simulink library "lib_AC_DFIG"  (R2026a)
settings: Solver=VariableStepAuto
undefined symbols (not defined in the file): block_buses, block_idx, buses_lf, fref, Lbiginv, Lrr_pu, Lss_pu, Nbuses, op_DFIG, Ps_lf, sigma
settings Model: Creator=atomas  LastModifiedBy=atomas

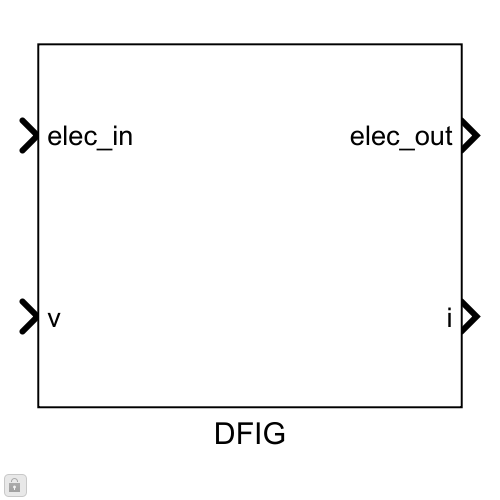
[thumbnail: Simulink's stored preview of the top-level diagram]
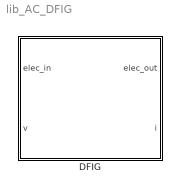
== system lib_AC_DFIG ==
  DFIG : Subsystem  mask(Doubly Fed Induction Generator){DFIGs_nodes=1, FBASE=50, D=0, H=3.3, Ls_pu=0.1178, Rs_pu=0.00734, Lm_pu=4.709, Rr_pu=0.01225, Lr_pu=0.15349, Ra_pu=0.1, La_pu=1, Cf_pu=0.0555, Ki_ia=7162, Kp_ia=6.5, Ki_ir=2117, Kp_ir=1.96, Ki_vc2=-562.5, Kp_vc2=-5.25, Ki_s=12000, Kp_s=1200, Kp_pll=2.33, Ki_pll=877}
      mask prompts: FBASE "Base frequency (Hz)"; D "Damping (pu)"; H "Inertia (s)"; Ls_pu "Stator inductances (pu)"; Rs_pu "Stator resistances (pu)"; Lm_pu "Mutual inductance (pu)"; Rr_pu "Rotor Resistance (pu)"; Lr_pu "Rotor Inductance"; Ra_pu "Filter Resistance (pu)"; La_pu "Filter Inductance (pu)"; Cf_pu "DC-Link Capacitance"; Ki_ia "GSC Ki"; Kp_ia "GSC Kp"; Ki_ir "RSC Ki"; Kp_ir "RSC Kp"; Ki_vc2 "DC Link Voltage Control Ki"; Kp_vc2 "DC Link Voltage Control Kp"; Ki_s "Slip Control Ki"; Kp_s "Slip Control Kp"; Kp_pll "PLL Kp"; Ki_pll "PLL Ki"
      mask help: Doubly Fed Induction Generator modelled in d-q reference frame.
      mask init:
      | [block_buses, block_idx, block_toM, block_fref, Lbiginv, Ls_pu, Lr_pu, Lm_pu, La_pu, Lss_pu, Lrr_pu, sigma, omega_base] = mask_init_DFIG(gcb, FBASE, Ls_pu, Lr_pu, Lm_pu, La_pu);
      mask Help: web([extractBefore(get_param(bdroot, 'filename'),gcs) 'Documentation/SM.html'])
      mask DialogControl Params Prompt: Parameters
      mask DialogControl Container10 Prompt: PI Parameters
      mask DialogControl Params_copy Prompt: Parameters

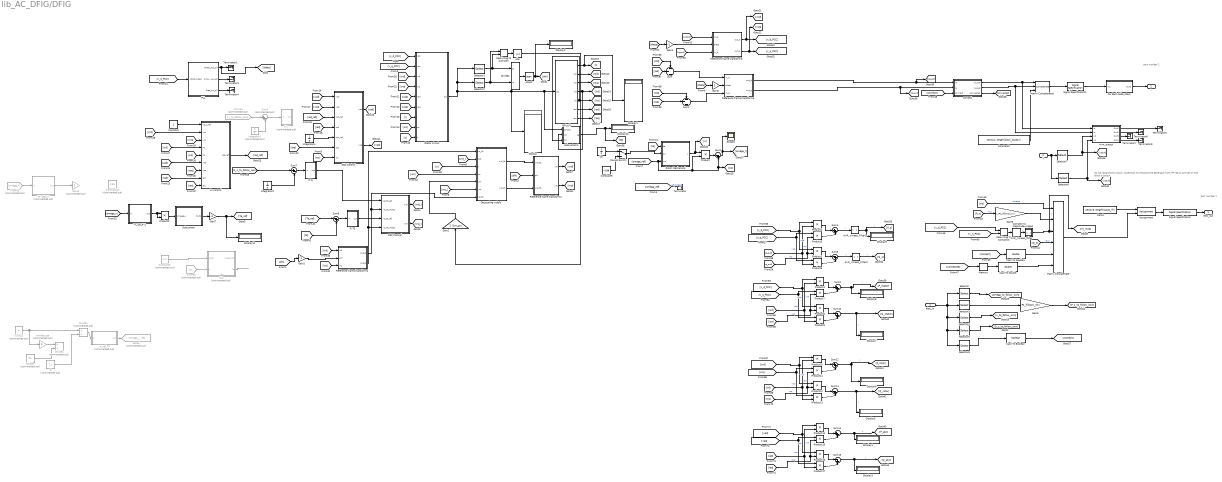
== system lib_AC_DFIG/DFIG ==
  note: do not rename this block, conditions to initialise the generator from PF result are set on this block's output
  note: port number 1
  note: port number 2
  elec_in : Inport
  v : Inport  Port=2
  AVR_Vmeas_Filter : Subsystem  mask{T_r=1e-6}
      mask prompts: T_r "Filter time constant"
      mask Display:
      | try
      |     dpoly(1, [T_r, 1])
      | catch
      | end
  AVR_Vmeas_Filter1 : Subsystem  mask{T_r=1e-6}
      mask prompts: T_r "Filter time constant"
      mask Display:
      | try
      |     dpoly(1, [T_r, 1])
      | catch
      | end
  AVR_Vmeas_Filter2 : Subsystem  mask{T_r=1e-6}
      mask prompts: T_r "Filter time constant"
      mask Display:
      | try
      |     dpoly(1, [T_r, 1])
      | catch
      | end
  Abs : Abs  SaturateOnIntegerOverflow=off
  Assignment : Assignment  NumberOfDimensions=2  DiagnosticForDimensions=Warning  IndexOptions=Assign all,Index vector (dialog)  Indices=1,block_idx  OutputSizes=1,1
  Atan2 : Trigonometry  SCDEnableBlockLinearizationSpecification=on  Operator=atan
  Cast To Boolean : DataTypeConversion  OutDataTypeStr=boolean  SaturateOnIntegerOverflow=off  RndMeth=Floor
  Cast To Double : DataTypeConversion  OutDataTypeStr=double  SaturateOnIntegerOverflow=off  RndMeth=Floor
  Cast To Double1 : DataTypeConversion  OutDataTypeStr=double  SaturateOnIntegerOverflow=off  RndMeth=Floor
  Complex to Magnitude-Angle1 : ComplexToMagnitudeAngle  Output=Magnitude
  Constant : Constant
  Constant10 : Constant  Commented=on  Value=1.83
  Constant2 : Constant  Value=zeros(1, length(block_buses))  VectorParams1D=off
  Constant6 : Constant  Commented=on  Value=-0.2
  Constant9 : Constant  Value=-0.89
  D : Constant  Commented=on  Value=11
  Decoupling vrdqFs : Subsystem
  Display{,1..11} (12 alike) : Display
  Divide1 : Product  Inputs=*/
  Divide2 : Product  Commented=on  Inputs=*/
  Divide4 : Product  Commented=on  Inputs=*/
  For Each Subsystem : Subsystem  TreatAsAtomicUnit=on
  From54 : From  Commented=on  GotoTag=v_to_follow_own
  From55 : From  Commented=on  GotoTag=omega_r
  From61 : From  Commented=on  GotoTag=s
  GSC Control : Subsystem
  Gain1 : Gain  Gain=-1
  Gain2 : Gain  Gain=1./Lm_pu
  Gain3 : Gain  Gain=Ps_lf(block_idx)
  Gain4 : Gain  Gain=-1
  Gain5 : Gain
  Gain6 : Gain  Commented=on  Gain=2
  Gain7 : Gain  Gain=-1
  Gain9 : Gain  Gain=1./Ps_lf(block_idx)
  Goto6 : Goto  Commented=on  GotoTag=omega_r_ref
  Integrator2 : Integrator  Commented=on  InitialCondition=op_DFIG.Integrator2
  Integrator3 : Integrator  InitialCondition=op_DFIG.Integrator3
  Integrator4 : Integrator  InitialCondition=op_DFIG.Integrator4
  Manual Switch : ManualSwitch
  Matrix Concatenate : Concatenate  NumInputs=6  Mode=Multidimensional array
  Matrix Concatenate1 : Concatenate  NumInputs=3  Mode=Multidimensional array
  Memory : Memory  InitialCondition=1
  PI Q : Subsystem
  PI TE : Subsystem
  PI v : Subsystem  Commented=on
  PLL : Subsystem
  Product{,1..17} (18 alike) : Product
  RSC Control : Subsystem
  Rblade : Constant  Commented=on  Value=28
  Real-Imag to Complex : RealImagToComplex
  Real-Imag to Complex3 : RealImagToComplex
  Reference frame transform2 : Subsystem
  Reference frame transform3 : Subsystem
  Reference frame transform4 : Subsystem
  Reference frame transform5 : Subsystem
  Rotor Mechanical : Subsystem
  Scope4 : Scope
      settings: ActiveDisplayYMinimum=0.94445  ActiveDisplayYMaximum=0.94472  DataLoggingVariableName=ScopeData2
  Selector : Selector  NumberOfDimensions=2  InputPortWidth=3  IndexOptions=Index vector (dialog),Index vector (dialog)  Indices=1,block_idx  OutputSizes=1,1
  Selector1 : Selector  NumberOfDimensions=2  InputPortWidth=9  IndexOptions=Index vector (dialog),Select all  Indices=2,1  OutputSizes=1,1
  Selector2 : Selector  NumberOfDimensions=2  InputPortWidth=9  IndexOptions=Index vector (dialog),Select all  Indices=1,1  OutputSizes=1,1
  Selector3 : Selector  NumberOfDimensions=2  InputPortWidth=3  IndexOptions=Index vector (dialog),Index vector (dialog)  Indices=2,block_idx  OutputSizes=1,1
  Selector4 : Selector  NumberOfDimensions=2  InputPortWidth=3  IndexOptions=Index vector (dialog),Index vector (dialog)  Indices=3,block_idx  OutputSizes=1,1
  Selector5 : Selector  NumberOfDimensions=2  InputPortWidth=3  IndexOptions=Index vector (dialog),Index vector (dialog)  Indices=4,block_idx  OutputSizes=1,1
  Selector6 : Selector  NumberOfDimensions=2  InputPortWidth=3  IndexOptions=Index vector (dialog),Index vector (dialog)  Indices=5,block_idx  OutputSizes=1,1
  Selector7 : Selector  NumberOfDimensions=2  InputPortWidth=3  IndexOptions=Index vector (dialog),Index vector (dialog)  Indices=1,block_buses  OutputSizes=1,1
  Selector8 : Selector  NumberOfDimensions=2  InputPortWidth=3  IndexOptions=Index vector (dialog),Index vector (dialog)  Indices=2,block_buses  OutputSizes=1,1
  Signal Specification : SignalSpecification  Dimensions=[6 length(buses_lf)]
  Signal Specification1 : SignalSpecification  Dimensions=[3 length(block_buses)]
  Slip : Subsystem  Commented=on
      settings: PortSchema="{\"entries\":[{\"content\":{\"sides\":[{\"content\":{\"connectorIds\":[\"In1\",\"In2\"]},\"type\":\"ConnectorPlacement.EquallySpacedRectSide\",\"uuid\":\"76dc537b-974c-49aa-a996-6680dce67c21\"},{\"content\":{\"connectorIds\":[\"Out1\",\"Out2\"],\"side\":\"RIGHT\"},\"type\":\"ConnectorPlacement.EquallySpacedRectSide\",\"uuid\":\"b6b8ef66-c2c7-4653-a511-fa1c360be79f\"},{\"content\":{\"connectorIds\":[],\"side\":\"TOP\"},\"type\":\"ConnectorPlacement.EquallySpacedRectSide\",\"uuid\":\"e58a1e6b-6a60-4748-900e-908d64e83c02\"},{\"content\":{\"connectorIds\":[\"In3\"],\"side\":\"BOTTOM\"},\"type\":\"ConnectorPlacement.EquallySpacedRectSide\",\"uuid\":\"479d910e-b2a0-4bf0-91fd-3472aae41677\"}]},\"type\":\"ConnectorPlacement.EquallySpacedConnector\",\"uuid\":\"d6647aa7-5f1b-4486-ad87-47217a09b45e\"}],\"packageUris\":[\"http://schema.mathworks.com/mf0/Connector/R2020b\"],\"version\":\"1.0\"}"
  Stator circuit : Subsystem
  Subsystem : Subsystem
  Subsystem1 : Subsystem
  Sum : Sum  Inputs=-|-|-
  Sum{1,5..6,10..11,13} (6 alike) : Sum  Inputs=|-+
  Sum{4,9,12,14} (4 alike) : Sum  Inputs=|++
  Sum2 : Sum  Inputs=-|-|-
  Sum3 : Sum  Commented=on  Inputs=|+-
  Sum7 : Sum  Inputs=|+-
  TF_DELAY : Subsystem  Commented=on  mask{T_s=0.0001}
      mask prompts: T_s "Filter time constant"
      mask Display:
      | try
      |     dpoly(1, [T_s, 1])
      | catch
      | end
  TF_DELAY1 : Subsystem  mask{T_s=20E-3}
      mask prompts: T_s "Filter time constant"
      mask Display:
      | try
      |     dpoly(1, [T_s, 1])
      | catch
      | end
  Terminator{,1,3..8} (8 alike) : Terminator
  Vc control : Subsystem
  Vwind1 : Constant  Commented=on  Value=6
  Zero1 : Constant  Value=zeros(6, length(buses_lf))  VectorParams1D=off  OutDataTypeStr=Inherit: Inherit via back propagation
  connect : Subsystem
  lambda_opt : Gain  Commented=on  Gain=8
  psi->i1 : Subsystem
  tm : Integrator  InitialCondition=op_DFIG.tm  LimitOutput=on  UpperSaturationLimit=0  LowerSaturationLimit=-1
  trim_output : Subsystem
  w_ref_TF : Subsystem  Commented=on  mask{T_s=0.05}
      mask prompts: T_s "Filter time constant"
      mask Display:
      | try
      |     dpoly(1, [T_s, 1])
      | catch
      | end
  elec_out : Outport
  i : Outport  Port=2
  wires:
  From61/1 -> Slip/2(s)
  TF_DELAY/1(out) -> Gain6/1
  From55/1 -> TF_DELAY/1(in)
  D/1 -> Divide4/2
  Subsystem1/1(te) -> [te], Display10/1
  Divide4/1 -> w_ref_TF/1(in)
  w_ref_TF/1(out) -> Goto6/1
  Rblade/1 -> Divide2/2
  lambda_opt/1 -> Divide2/1
  Vwind1/1 -> Divide4/1, lambda_opt/1
  Sum7/1 -> PI Q/1(in)
  Sum4/1 -> AVR_Vmeas_Filter1/1(in)  "v"
  Sum5/1 -> AVR_Vmeas_Filter2/1(in)  "v"
  Real-Imag to Complex3/1 -> Complex to Magnitude-Angle1/1
  [v_q_PCC] -> Real-Imag to Complex3/2
  Complex to Magnitude-Angle1/1 -> AVR_Vmeas_Filter/1(in)  "v"
  [v_d_PCC] -> Real-Imag to Complex3/1
  Product5/1 -> Sum5/1
  [v_d_PCC] -> Product1/1, Product5/1  "vod"
  Product3/1 -> Sum4/2
  [id_out] -> Product1/2, Product6/2  "iod"
  [v_q_PCC] -> Product6/1, Product3/1  "voq"
  Product6/1 -> Sum5/2
  Product1/1 -> Sum4/1
  [iq_out] -> Product3/2, Product5/2  "ioq"
  tm/1 -> Manual Switch/1
  Signal Specification/1 -> elec_out/1
  Gain4/1 -> Reference frame transform3/2(theta)
  [vaq] -> Stator circuit/6(vaq)
  Constant9/1 -> Manual Switch/2
  Sum/1 -> Reference frame transform5/1(in_d)
  Sum2/1 -> Reference frame transform5/3(in_q)
  PLL/1(theta_rad_pll) -> [theta], Terminator1/1
  For Each Subsystem/1(Out1) -> i/1
  Reference frame transform5/1(out_d) -> connect/1(id), [id_out]
  Product/1 -> Sum1/1
  [v_d_PCC] -> Stator circuit/1(vsd)
  trim_output/2(Out2) -> Terminator6/1
  ? -> Sum2/3
  [vrd_] -> Decoupling vrdqFs/2(Vrd')
  [vad] -> Stator circuit/5(vad)
  Selector5/1 -> [Q_s_to_follow_own]
  [iad] -> GSC Control/4(iad)
  Vc control/1(iad_ref) -> [iad_ref]
  psi->i1/5(irq) -> [irq], Subsystem1/3(irq)
  Real-Imag to Complex/1 -> Abs/1
  [vrd] -> Vc control/2(vrd)
  [vad] -> Vc control/6(vad)
  [te] -> Rotor Mechanical/1(te)
  [omega_ref] -> Terminator/1  "ref_omega"
  [vrd] -> Stator circuit/3(vrd)
  Assignment/1 -> Signal Specification/1
  Reference frame transform2/2(vrq) -> [vrq]
  [v_q_PCC] -> PLL/1(vdq0_meas)
  Decoupling vrdqFs/1(vrd_Fs) -> Reference frame transform2/1(vrd_Fs)
  GSC Control/1(vad) -> [vad]
  [v_q_PCC] -> Stator circuit/2(vsq)
  psi->i1/6(iad) -> [iad]
  [iaq] -> Vc control/9(iaq)
  Selector2/1 -> Divide1/2, Real-Imag to Complex/1
  GSC Control/2(vaq) -> [vaq]
  [vsq] -> GSC Control/2(vsq)
  RSC Control/2(vrq') -> [vrq_]
  RSC Control/1(vrd') -> [vrd_]
  [phi] -> Gain1/1
  [vrq] -> Vc control/3(vrq)
  Divide1/1 -> Atan2/1
  [ws] -> Decoupling vrdqFs/4(ws)
  Reference frame transform2/1(vrd) -> [vrd]
  PLL/2(omega_pu_pll) -> Terminator3/1
  [vrq_] -> Decoupling vrdqFs/6(vrq')
  psi->i1/3(isq) -> [isq]
  [iad_ref] -> GSC Control/3(iad_ref)
  ? -> Sum/3
  PLL/3(Freq_Hz_pll) -> Terminator4/1
  Constant/1 -> Vc control/1(Vc_2_ref)
  [iad] -> Vc control/8(iad)
  Gain2/1 -> Decoupling vrdqFs/5(ism)
  [vdout] -> Reference frame transform3/1(in_d)
  [theta] -> Gain4/1
  Gain9/1 -> Matrix Concatenate/2
  Reference frame transform3/2(out_q) -> [vsq], [v_q_PCC]
  [P_s] -> Gain9/1  "P_s"
  [isd] -> Sum/1
  psi->i1/4(ird) -> [ird], Subsystem1/2(ird)
  Matrix Concatenate1/1 -> Signal Specification1/1
  trim_output/4(Out4) -> Terminator8/1
  Selector8/1 -> [vqout], trim_output/4(vq)
  Constant2/1 -> Matrix Concatenate1/3
  [irq] -> Reference frame transform4/3(irq)
  [vqout] -> Reference frame transform3/3(in_q)
  trim_output/3(Out3) -> Terminator7/1
  Cast To Boolean/1 -> [connect]
  [ws] -> Stator circuit/8(ws)
  v/1 -> Selector8/1, Selector7/1
  Rotor Mechanical/1(s) -> Product/1, [s]
  [i] -> Stator circuit/7(i)
  Signal Specification1/1 -> For Each Subsystem/1(In1)
  [vsd] -> GSC Control/1(vsd)
  Reference frame transform4/2(out_q) -> RSC Control/4(irq_Fs_meas), Decoupling vrdqFs/1(irq_Fs)
  Atan2/1 -> [phi], Display2/1
  [ws] -> GSC Control/7(ws)
  Selector7/1 -> trim_output/3(vd), [vdout]
  Gain5/1 -> Reference frame transform5/2(theta)
  elec_in/1 -> Selector6/1, Selector5/1, Selector4/1, Selector3/1, Selector/1
  connect/2(iq_real) -> trim_output/2(iq), Matrix Concatenate1/2
  [connect] -> Cast To Double1/1
  Cast To Double/1 -> Matrix Concatenate/6
  Cast To Double1/1 -> Matrix Concatenate/5
  [phi] -> Reference frame transform2/2(phi)
  Selector6/1 -> Cast To Boolean/1
  [Q_s] -> Matrix Concatenate/4  "Q_s"
  connect/1(id_real) -> trim_output/1(id), Matrix Concatenate1/1
  [ird] -> Reference frame transform4/1(ird)
  psi->i1/7(iaq) -> [iaq]
  [vrq] -> Stator circuit/4(vrq)
  psi->i1/1(i) -> Display1/1, [i]
  trim_output/1(Out1) -> Terminator5/1
  [ws] -> Matrix Concatenate/1  "omega"
  Zero1/1 -> Assignment/1
  Selector/1 -> [omega_to_follow_own]
  Selector3/1 -> Gain3/1
  Selector4/1 -> [v_to_follow_own]
  Gain3/1 -> [P_s_to_follow_own]
  [vaq] -> Vc control/7(vaq)
  [ird] -> Vc control/4(ird)
  Matrix Concatenate/1 -> Assignment/2
  [iaq] -> GSC Control/6(iaq)
  [isq] -> Sum2/1
  [omega_ref] -> Rotor Mechanical/3(ws), Product/2, [ws], Sum1/2
  Reference frame transform5/2(out_q) -> connect/2(iq), [iq_out]
  [theta] -> Gain5/1
  psi->i1/2(isd) -> [isd]
  Stator circuit/1(psi) -> Display/1, psi->i1/1(psi), Subsystem1/1(psisdq), Selector1/1, Selector2/1
  [connect] -> connect/3(connect)
  [s] -> Stator circuit/9(s)
  Decoupling vrdqFs/2(vrq_Fs) -> Reference frame transform2/3(vrq_Fs)
  Reference frame transform3/1(out_d) -> [vsd], [v_d_PCC]
  [s] -> Decoupling vrdqFs/3(s)
  [iad] -> Sum/2
  AVR_Vmeas_Filter/1(out) -> [Vt_mod], Matrix Concatenate/3  "v"
  Selector1/1 -> Divide1/1, Real-Imag to Complex/2
  [connected] -> Memory/1
  [irq] -> Vc control/5(irq)
  connect/3(connected) -> [connected]
  [iaq] -> Sum2/2
  Gain1/1 -> Reference frame transform4/2(phi)
  Memory/1 -> Cast To Double/1
  [isd] -> Product4/2, Product9/2  "iod"
  [isq] -> Product7/2, Product8/2  "ioq"
  Product9/1 -> Sum10/2
  Product7/1 -> Sum9/2
  [v_d_PCC] -> Product4/1, Product8/1  "vod"
  Sum10/1 -> [Q_stator], Display7/1  "v"
  [v_q_PCC] -> Product9/1, Product7/1  "voq"
  Product4/1 -> Sum9/1
  Sum9/1 -> Display8/1, [P_stator]  "v"
  Product8/1 -> Sum10/1
  Product12/1 -> Sum11/1
  Sum12/1 -> [P_rotor], Display6/1  "v"
  Product10/1 -> Sum12/1
  [vrq] -> Product11/1, Product13/1  "voq"
  Sum11/1 -> Display5/1, [Q_rotor]  "v"
  [vrd] -> Product12/1, Product10/1  "vod"
  Product11/1 -> Sum12/2
  Product13/1 -> Sum11/2
  [irq] -> Product12/2, Product11/2  "ioq"
  [ird] -> Product13/2, Product10/2  "iod"
  [iad] -> Product14/2, Product17/2  "iod"
  [iaq] -> Product15/2, Product16/2  "ioq"
  Product17/1 -> Sum13/2
  Product15/1 -> Sum14/2
  [vad] -> Product14/1, Product16/1  "vod"
  Sum13/1 -> [Q_gsc], Display3/1  "v"
  [vaq] -> Product17/1, Product15/1  "voq"
  Product14/1 -> Sum14/1
  Sum14/1 -> Display4/1, [P_gsc]  "v"
  Product16/1 -> Sum13/1
  Constant6/1 -> Slip/1(s_ref)
  Slip/2(Te) -> ?
  Integrator3/1 -> Sum7/2
  AVR_Vmeas_Filter1/1(out) -> [P_s], Display9/1  "v"
  AVR_Vmeas_Filter2/1(out) -> [Q_s]  "v"
  Subsystem/1(Out1) -> Gain7/1
  Product2/1 -> Subsystem/1(omega_r)
  [omega_r] -> TF_DELAY1/1(in)
  Sum3/1 -> PI v/1(in)
  From54/1 -> Sum3/1
  Sum1/1 -> [omega_r], Scope4/1
  Abs/1 -> Gain2/1
  Integrator2/1 -> Sum3/2
  Gain7/1 -> Display11/1, [Te_ref]
  [Te_ref] -> Sum6/1
  [te] -> Sum6/2
  Sum6/1 -> PI TE/1(in)
  TF_DELAY1/1(out) -> Product2/2, Product2/1
  [Q_s_to_follow_own] -> Sum7/1
  Integrator4/1 -> GSC Control/5(iaq_ref)
  PI TE/1(out) -> RSC Control/3(irq_Fs_ref)
  Reference frame transform4/1(out_d) -> RSC Control/2(ird_Fs_meas), Decoupling vrdqFs/7(ird_Fs)
  PI Q/1(out) -> RSC Control/1(ird_Fs_ref)
  Manual Switch/1 -> Rotor Mechanical/2(tm)

== system lib_AC_DFIG/DFIG/AVR_Vmeas_Filter ==
  in : Inport
  Gain : Gain  Gain=1./T_r
  Sum4 : Sum  Inputs=|+-
  x_a : Integrator  InitialCondition=op_DFIG.AVR_Vmeas_Filter_x_a
  out : Outport
  wires:
  x_a/1 -> Sum4/2, out/1
  in/1 -> Sum4/1
  Sum4/1 -> Gain/1
  Gain/1 -> x_a/1

== system lib_AC_DFIG/DFIG/AVR_Vmeas_Filter1 ==
  in : Inport
  Gain : Gain  Gain=1./T_r
  Sum4 : Sum  Inputs=|+-
  x_a : Integrator  InitialCondition=op_DFIG.AVR_Vmeas_Filter1_x_a
  out : Outport
  wires:
  Gain/1 -> x_a/1
  Sum4/1 -> Gain/1
  in/1 -> Sum4/1
  x_a/1 -> out/1, Sum4/2

== system lib_AC_DFIG/DFIG/AVR_Vmeas_Filter2 ==
  in : Inport
  Gain : Gain  Gain=1./T_r
  Sum4 : Sum  Inputs=|+-
  x_a : Integrator  InitialCondition=op_DFIG.AVR_Vmeas_Filter2_x_a
  out : Outport
  wires:
  x_a/1 -> Sum4/2, out/1
  in/1 -> Sum4/1
  Sum4/1 -> Gain/1
  Gain/1 -> x_a/1

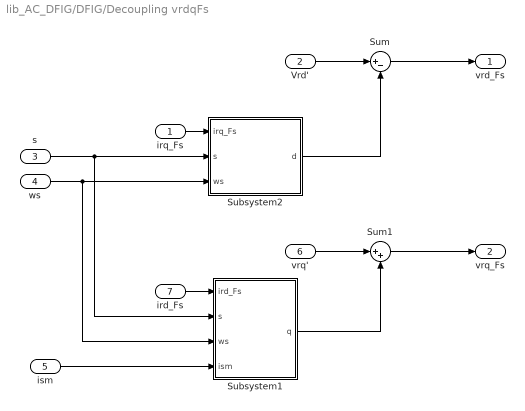
== system lib_AC_DFIG/DFIG/Decoupling vrdqFs ==
  irq_Fs : Inport
  Vrd' : Inport  Port=2
  s : Inport  Port=3
  ws : Inport  Port=4
  ism : Inport  Port=5
  vrq' : Inport  Port=6
  ird_Fs : Inport  Port=7
  Subsystem1 : Subsystem
  Subsystem2 : Subsystem
  Sum : Sum  Inputs=|+-
  Sum1 : Sum  Inputs=|++
  vrd_Fs : Outport
  vrq_Fs : Outport  Port=2
  wires:
  vrq'/1 -> Sum1/1
  ird_Fs/1 -> Subsystem1/1(ird_Fs)
  irq_Fs/1 -> Subsystem2/1(irq_Fs)
  Sum/1 -> vrd_Fs/1
  Vrd'/1 -> Sum/1
  s/1 -> Subsystem2/2(s), Subsystem1/2(s)
  ws/1 -> Subsystem2/3(ws), Subsystem1/3(ws)
  Subsystem2/1(d) -> Sum/2
  Subsystem1/1(q) -> Sum1/2
  Sum1/1 -> vrq_Fs/1
  ism/1 -> Subsystem1/4(ism)

== system lib_AC_DFIG/DFIG/For Each Subsystem ==
  In1 : Inport  Partition=on  PartitionDimension=1  PartitionWidth=1  PartitionOffset=0
  Assignment : Assignment  DiagnosticForDimensions=Warning  IndexOptions=Index vector (dialog)  Indices=block_buses  OutputSizes=1
  For Each : ForEach  DisableCoverage=on
  Zero : Constant  Value=zeros(1,Nbuses)  VectorParams1D=off  OutDataTypeStr=Inherit: Inherit via back propagation
  Out1 : Outport  ConcatenationDimension=1
  wires:
  Assignment/1 -> Out1/1
  In1/1 -> Assignment/2
  Zero/1 -> Assignment/1

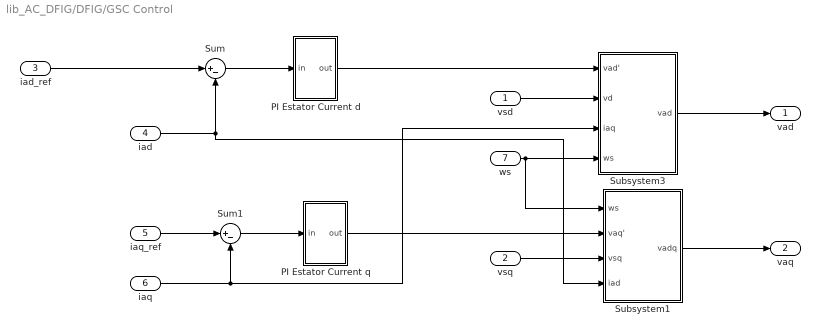
== system lib_AC_DFIG/DFIG/GSC Control ==
  vsd : Inport
  vsq : Inport  Port=2
  iad_ref : Inport  Port=3
  iad : Inport  Port=4
  iaq_ref : Inport  Port=5
  iaq : Inport  Port=6
  ws : Inport  Port=7
  PI Estator Current d : Subsystem
  PI Estator Current q : Subsystem
  Subsystem1 : Subsystem
  Subsystem3 : Subsystem
  Sum : Sum  Inputs=|+-
  Sum1 : Sum  Inputs=|+-
  vad : Outport  VectorParamsAs1DForOutWhenUnconnected=off
  vaq : Outport  Port=2  VectorParamsAs1DForOutWhenUnconnected=off
  wires:
  Subsystem1/1(vadq) -> vaq/1
  vsq/1 -> Subsystem1/3(vsq)
  ws/1 -> Subsystem3/4(ws), Subsystem1/1(ws)
  iaq/1 -> Sum1/2, Subsystem3/3(iaq)
  iaq_ref/1 -> Sum1/1
  iad_ref/1 -> Sum/1
  Sum/1 -> PI Estator Current d/1(in)
  Sum1/1 -> PI Estator Current q/1(in)
  iad/1 -> Subsystem1/4(iad), Sum/2
  PI Estator Current d/1(out) -> Subsystem3/1(vad')
  PI Estator Current q/1(out) -> Subsystem1/2(vaq')
  vsd/1 -> Subsystem3/2(vd)
  Subsystem3/1(vad) -> vad/1

== system lib_AC_DFIG/DFIG/PI Q ==
  in : Inport
  Gain : Gain  Gain=0.25
  Gain1 : Gain  Gain=0.5
  Gain2 : Gain
  Gain3 : Gain
  Sum : Sum  Inputs=++|
  pi q : Integrator  InitialCondition=op_DFIG.PI_Q_pi_q  UpperSaturationLimit=1.01  LowerSaturationLimit=0.99
  out : Outport  VectorParamsAs1DForOutWhenUnconnected=off
  wires:
  pi q/1 -> Sum/2
  Gain/1 -> Gain2/1
  in/1 -> Gain/1, Gain1/1
  Sum/1 -> out/1
  Gain1/1 -> Gain3/1
  Gain2/1 -> Sum/1
  Gain3/1 -> pi q/1

== system lib_AC_DFIG/DFIG/PI TE ==
  in : Inport
  Gain : Gain  Gain=0.25
  Gain1 : Gain  Gain=0.5
  Gain2 : Gain
  Gain3 : Gain
  Sum : Sum  Inputs=++|
  pi TE : Integrator  InitialCondition=op_DFIG.PI_TE_pi_TE  UpperSaturationLimit=1.01  LowerSaturationLimit=0.99
  out : Outport  VectorParamsAs1DForOutWhenUnconnected=off
  wires:
  Gain1/1 -> Gain3/1
  Gain2/1 -> Sum/1
  Sum/1 -> out/1
  in/1 -> Gain1/1, Gain/1
  Gain/1 -> Gain2/1
  pi TE/1 -> Sum/2
  Gain3/1 -> pi TE/1

== system lib_AC_DFIG/DFIG/PI v ==
  in : Inport
  Gain : Gain  Gain=0.25
  Gain1 : Gain  Gain=0.5
  Gain2 : Gain
  Gain3 : Gain
  Gain4 : Gain  Gain=0.000001
  Sum : Sum  Inputs=++|
  pi q : Integrator  InitialCondition=op_DFIG.PI_v_pi_q  UpperSaturationLimit=1.01  LowerSaturationLimit=0.99
  out : Outport  VectorParamsAs1DForOutWhenUnconnected=off
  wires:
  Gain3/1 -> pi q/1
  Gain2/1 -> Sum/1
  Gain1/1 -> Gain3/1
  Sum/1 -> out/1
  in/1 -> Gain4/1
  Gain/1 -> Gain2/1
  pi q/1 -> Sum/2
  Gain4/1 -> Gain/1, Gain1/1

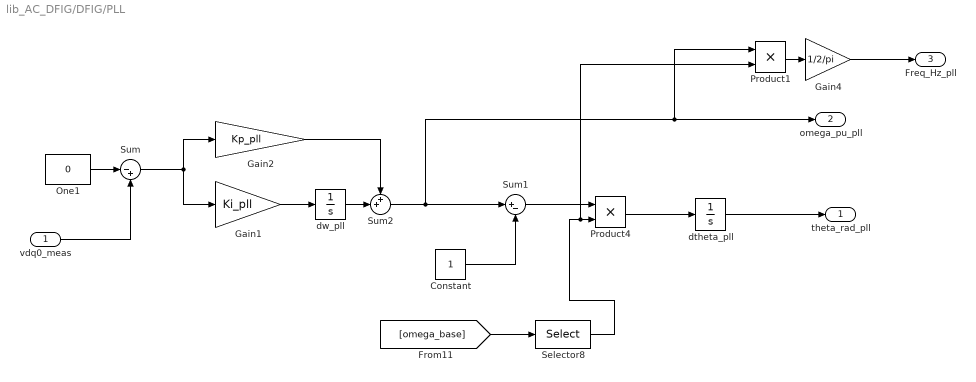
== system lib_AC_DFIG/DFIG/PLL ==
  vdq0_meas : Inport
  Constant : Constant
  Gain1 : Gain  Gain=Ki_pll
  Gain2 : Gain  Gain=Kp_pll
  Gain4 : Gain  Gain=1/2/pi
  One1 : Constant  Value=0  OutDataTypeStr=Inherit: Inherit via back propagation
  Product1 : Product
  Product4 : Product
  Selector8 : Selector  InputPortWidth=length(fref.ref_units)  IndexOptions=Index vector (dialog)  Indices=block_fref  OutputSizes=1
  Sum : Sum  Inputs=|-+
  Sum1 : Sum  Inputs=|+-
  Sum2 : Sum  Inputs=++|
  dtheta_pll : Integrator  InitialCondition=op_DFIG.PLL_dtheta_pll
  dw_pll : Integrator  InitialCondition=op_DFIG.PLL_dw_pll
  theta_rad_pll : Outport
  omega_pu_pll : Outport  Port=2
  Freq_Hz_pll : Outport  Port=3
  wires:
  One1/1 -> Sum/1
  vdq0_meas/1 -> Sum/2
  Gain4/1 -> Freq_Hz_pll/1
  dw_pll/1 -> Sum2/2
  Gain2/1 -> Sum2/1
  Sum/1 -> Gain2/1, Gain1/1
  Gain1/1 -> dw_pll/1
  dtheta_pll/1 -> theta_rad_pll/1
  Product1/1 -> Gain4/1
  Sum2/1 -> Sum1/1, Product1/1, omega_pu_pll/1
  Sum1/1 -> Product4/1
  Constant/1 -> Sum1/2
  Product4/1 -> dtheta_pll/1
  Selector8/1 -> Product1/2, Product4/2
  [omega_base] -> Selector8/1

== system lib_AC_DFIG/DFIG/RSC Control ==
  ird_Fs_ref : Inport
  ird_Fs_meas : Inport  Port=2
  irq_Fs_ref : Inport  Port=3
  irq_Fs_meas : Inport  Port=4
  PI Rotor Current d : Subsystem
  PI Rotor Current q : Subsystem
  Sum : Sum  Inputs=|+-
  Sum1 : Sum  Inputs=|+-
  vrd' : Outport  VectorParamsAs1DForOutWhenUnconnected=off
  vrq' : Outport  Port=2  VectorParamsAs1DForOutWhenUnconnected=off
  wires:
  Sum1/1 -> PI Rotor Current q/1(in)
  irq_Fs_ref/1 -> Sum1/1
  irq_Fs_meas/1 -> Sum1/2
  ird_Fs_meas/1 -> Sum/2
  PI Rotor Current q/1(out) -> vrq'/1
  PI Rotor Current d/1(out) -> vrd'/1
  Sum/1 -> PI Rotor Current d/1(in)
  ird_Fs_ref/1 -> Sum/1

== system lib_AC_DFIG/DFIG/Reference frame transform2 ==
  vrd_Fs : Inport
  phi : Inport  Port=2
  vrq_Fs : Inport  Port=3
  Complex to Real-Imag : ComplexToRealImag
  Cos : Trigonometry  SCDEnableBlockLinearizationSpecification=on  Operator=cos
  Product : Product
  Real-Imag to Complex : RealImagToComplex
  Real-Imag to Complex1 : RealImagToComplex
  Sin : Trigonometry  SCDEnableBlockLinearizationSpecification=on
  vrd : Outport
  vrq : Outport  Port=2
  wires:
  Complex to Real-Imag/2 -> vrq/1
  Real-Imag to Complex1/1 -> Product/1
  Real-Imag to Complex/1 -> Product/2
  Product/1 -> Complex to Real-Imag/1
  phi/1 -> Sin/1, Cos/1
  Cos/1 -> Real-Imag to Complex1/1
  Sin/1 -> Real-Imag to Complex1/2
  Complex to Real-Imag/1 -> vrd/1
  vrq_Fs/1 -> Real-Imag to Complex/2
  vrd_Fs/1 -> Real-Imag to Complex/1

== system lib_AC_DFIG/DFIG/Reference frame transform3 ==
  in_d : Inport
  theta : Inport  Port=2
  in_q : Inport  Port=3
  Complex to Real-Imag : ComplexToRealImag
  Cos : Trigonometry  SCDEnableBlockLinearizationSpecification=on  Operator=cos
  Product : Product
  Real-Imag to Complex : RealImagToComplex
  Real-Imag to Complex1 : RealImagToComplex
  Sin : Trigonometry  SCDEnableBlockLinearizationSpecification=on
  out_d : Outport
  out_q : Outport  Port=2
  wires:
  Complex to Real-Imag/2 -> out_q/1
  Real-Imag to Complex1/1 -> Product/1
  Real-Imag to Complex/1 -> Product/2
  Product/1 -> Complex to Real-Imag/1
  theta/1 -> Sin/1, Cos/1
  Cos/1 -> Real-Imag to Complex1/1
  Sin/1 -> Real-Imag to Complex1/2
  Complex to Real-Imag/1 -> out_d/1
  in_q/1 -> Real-Imag to Complex/2
  in_d/1 -> Real-Imag to Complex/1

== system lib_AC_DFIG/DFIG/Reference frame transform4 ==
  ird : Inport
  phi : Inport  Port=2
  irq : Inport  Port=3
  Complex to Real-Imag : ComplexToRealImag
  Cos : Trigonometry  SCDEnableBlockLinearizationSpecification=on  Operator=cos
  Product : Product
  Real-Imag to Complex : RealImagToComplex
  Real-Imag to Complex1 : RealImagToComplex
  Sin : Trigonometry  SCDEnableBlockLinearizationSpecification=on
  out_d : Outport
  out_q : Outport  Port=2
  wires:
  ird/1 -> Real-Imag to Complex/1
  irq/1 -> Real-Imag to Complex/2
  Complex to Real-Imag/1 -> out_d/1
  Sin/1 -> Real-Imag to Complex1/2
  Cos/1 -> Real-Imag to Complex1/1
  phi/1 -> Cos/1, Sin/1
  Product/1 -> Complex to Real-Imag/1
  Real-Imag to Complex/1 -> Product/2
  Real-Imag to Complex1/1 -> Product/1
  Complex to Real-Imag/2 -> out_q/1

== system lib_AC_DFIG/DFIG/Reference frame transform5 ==
  in_d : Inport
  theta : Inport  Port=2
  in_q : Inport  Port=3
  Complex to Real-Imag : ComplexToRealImag
  Cos : Trigonometry  SCDEnableBlockLinearizationSpecification=on  Operator=cos
  Product : Product
  Real-Imag to Complex : RealImagToComplex
  Real-Imag to Complex1 : RealImagToComplex
  Sin : Trigonometry  SCDEnableBlockLinearizationSpecification=on
  out_d : Outport
  out_q : Outport  Port=2
  wires:
  in_d/1 -> Real-Imag to Complex/1
  in_q/1 -> Real-Imag to Complex/2
  Complex to Real-Imag/1 -> out_d/1
  Sin/1 -> Real-Imag to Complex1/2
  Cos/1 -> Real-Imag to Complex1/1
  theta/1 -> Cos/1, Sin/1
  Product/1 -> Complex to Real-Imag/1
  Real-Imag to Complex/1 -> Product/2
  Real-Imag to Complex1/1 -> Product/1
  Complex to Real-Imag/2 -> out_q/1

== system lib_AC_DFIG/DFIG/Rotor Mechanical ==
  te : Inport
  tm : Inport  Port=2
  ws : Inport  Port=3
  Divide : Product  Inputs=*/
  Gain : Gain  Gain=1./(2*H)
  Gain1 : Gain  Gain=0.01
  Sum1 : Sum  Inputs=+|-|-  InputSameDT=on  SaturateOnIntegerOverflow=on  OutDataTypeStr=Inherit: Same as first input
  slip : Integrator  InitialCondition=op_DFIG.Rotor_Mechanical_slip  UpperSaturationLimit=1.3  LowerSaturationLimit=0.7
  s : Outport  VectorParamsAs1DForOutWhenUnconnected=off
  wires:
  Gain1/1 -> Sum1/3
  Sum1/1 -> Gain/1
  te/1 -> Sum1/2
  tm/1 -> Sum1/1
  Gain/1 -> Divide/1
  Divide/1 -> slip/1  "ds"
  ws/1 -> Divide/2
  slip/1 -> Gain1/1, s/1

== system lib_AC_DFIG/DFIG/Slip ==
  s_ref : Inport
  s : Inport  Port=2
  Fs : Inport  Port=3
  Gain : Gain  Gain=-1
  Gain1 : Gain  Gain=Lm_pu./Lss_pu
  PI Slip : Subsystem
  Product : Product
  Sum : Sum  Inputs=|+-
  irq_Fs_ref : Outport  VectorParamsAs1DForOutWhenUnconnected=off
  Te : Outport  Port=2  VectorParamsAs1DForOutWhenUnconnected=off
  wires:
  s_ref/1 -> Sum/1
  s/1 -> Sum/2
  PI Slip/1(out) -> Product/1, irq_Fs_ref/1
  Sum/1 -> PI Slip/1(in)
  Gain/1 -> Product/2
  Product/1 -> Gain1/1
  Gain1/1 -> Te/1
  Fs/1 -> Gain/1

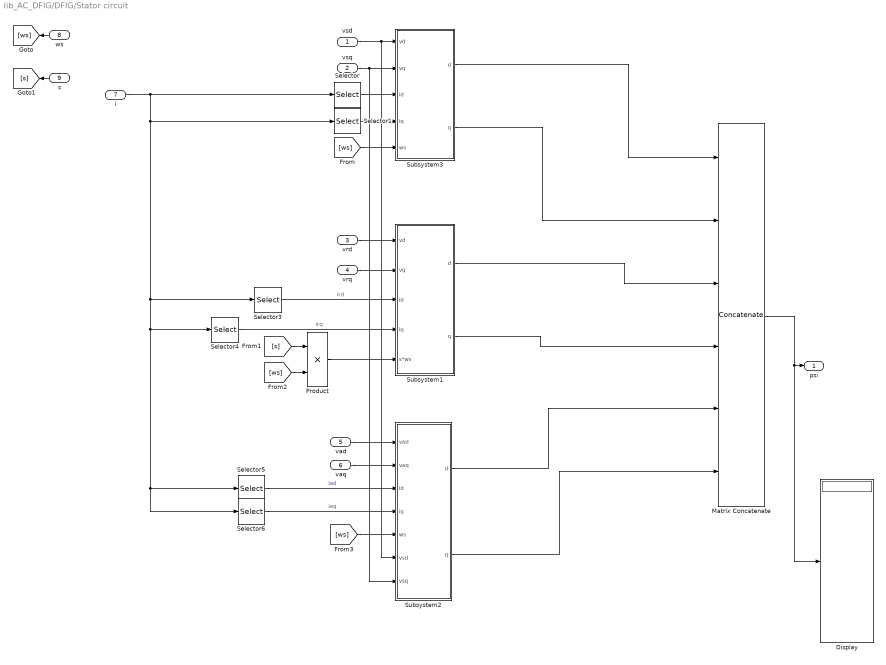
== system lib_AC_DFIG/DFIG/Stator circuit ==
  vsd : Inport
  vsq : Inport  Port=2
  vrd : Inport  Port=3
  vrq : Inport  Port=4
  vad : Inport  Port=5
  vaq : Inport  Port=6
  i : Inport  Port=7
  ws : Inport  Port=8
  s : Inport  Port=9
  Display : Display
  Matrix Concatenate : Concatenate  NumInputs=6  Mode=Multidimensional array
  Product : Product
  Selector : Selector  NumberOfDimensions=2  InputPortWidth=9  IndexOptions=Index vector (dialog),Select all  Indices=[1],1  OutputSizes=1,1
  Selector1 : Selector  NumberOfDimensions=2  InputPortWidth=9  IndexOptions=Index vector (dialog),Select all  Indices=[2],1  OutputSizes=1,1
  Selector3 : Selector  NumberOfDimensions=2  InputPortWidth=9  IndexOptions=Index vector (dialog),Select all  Indices=3,1  OutputSizes=1,1
  Selector4 : Selector  NumberOfDimensions=2  InputPortWidth=9  IndexOptions=Index vector (dialog),Select all  Indices=4,1  OutputSizes=1,1
  Selector5 : Selector  NumberOfDimensions=2  InputPortWidth=9  IndexOptions=Index vector (dialog),Select all  Indices=5,1  OutputSizes=1,1
  Selector6 : Selector  NumberOfDimensions=2  InputPortWidth=9  IndexOptions=Index vector (dialog),Select all  Indices=6,1  OutputSizes=1,1
  Subsystem1 : Subsystem
  Subsystem2 : Subsystem
  Subsystem3 : Subsystem
  psi : Outport  VectorParamsAs1DForOutWhenUnconnected=off
  wires:
  Matrix Concatenate/1 -> Display/1, psi/1
  Selector6/1 -> Subsystem2/4(iq)  "iaq"
  Selector5/1 -> Subsystem2/3(id)  "iad"
  Subsystem1/2(q) -> Matrix Concatenate/4
  Subsystem1/1(d) -> Matrix Concatenate/3
  vaq/1 -> Subsystem2/2(vaq)
  vad/1 -> Subsystem2/1(vad)
  Selector4/1 -> Subsystem1/4(iq)  "irq"
  Selector3/1 -> Subsystem1/3(id)  "ird"
  Product/1 -> Subsystem1/5(s*ws)
  vrq/1 -> Subsystem1/2(vq)
  vrd/1 -> Subsystem1/1(vd)
  [ws] -> Subsystem3/5(ws)
  Subsystem3/2(q) -> Matrix Concatenate/2
  Subsystem3/1(d) -> Matrix Concatenate/1
  Selector/1 -> Subsystem3/3(id)
  Selector1/1 -> Subsystem3/4(iq)
  vsq/1 -> Subsystem2/7(vsq), Subsystem3/2(vq)
  vsd/1 -> Subsystem2/6(vsd), Subsystem3/1(vd)
  [ws] -> Product/2
  s/1 -> [s]
  ws/1 -> [ws]
  i/1 -> Selector/1, Selector1/1, Selector5/1, Selector6/1, Selector4/1, Selector3/1
  [s] -> Product/1
  [ws] -> Subsystem2/5(ws)
  Subsystem2/1(d) -> Matrix Concatenate/5
  Subsystem2/2(q) -> Matrix Concatenate/6

== system lib_AC_DFIG/DFIG/Subsystem ==
  note: 10.1109/PES.2008.4596214
  omega_r : Inport
  Gain1 : Gain  Commented=on  Gain=0.5896
  Gain2 : Gain  Gain=0.5787
  Out1 : Outport
  wires:
  Gain2/1 -> Out1/1
  omega_r/1 -> Gain2/1

== system lib_AC_DFIG/DFIG/Subsystem1 ==
  psisdq : Inport
  ird : Inport  Port=2
  irq : Inport  Port=3
  Product4 : Product
  Product7 : Product
  Selector1 : Selector  NumberOfDimensions=2  InputPortWidth=6  IndexOptions=Index vector (dialog),Select all  Indices=3,1  OutputSizes=1,1
  Selector10 : Selector  NumberOfDimensions=2  InputPortWidth=6  IndexOptions=Index vector (dialog),Select all  Indices=4,1  OutputSizes=1,1
  Sum8 : Sum  Inputs=|+-
  te : Outport
  wires:
  Product7/1 -> Sum8/2
  ird/1 -> Product4/2
  Product4/1 -> Sum8/1
  Selector1/1 -> Product7/1
  Selector10/1 -> Product4/1
  psisdq/1 -> Selector10/1, Selector1/1
  irq/1 -> Product7/2
  Sum8/1 -> te/1

== system lib_AC_DFIG/DFIG/TF_DELAY ==
  in : Inport
  Gain : Gain  Gain=1./T_s
  Sum4 : Sum  Inputs=|+-
  x_a : Integrator  InitialCondition=op_DFIG.TF_DELAY_x_a
  out : Outport
  wires:
  Gain/1 -> x_a/1
  Sum4/1 -> Gain/1
  x_a/1 -> out/1, Sum4/2
  in/1 -> Sum4/1

== system lib_AC_DFIG/DFIG/TF_DELAY1 ==
  in : Inport
  Gain : Gain  Gain=1./T_s
  Sum4 : Sum  Inputs=|+-
  x_a : Integrator  InitialCondition=op_DFIG.TF_DELAY1_x_a
  out : Outport
  wires:
  in/1 -> Sum4/1
  x_a/1 -> Sum4/2, out/1
  Sum4/1 -> Gain/1
  Gain/1 -> x_a/1

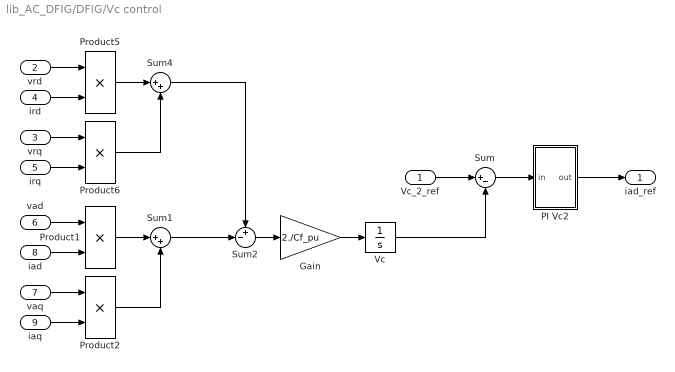
== system lib_AC_DFIG/DFIG/Vc control ==
  Vc_2_ref : Inport
  vrd : Inport  Port=2
  vrq : Inport  Port=3
  ird : Inport  Port=4
  irq : Inport  Port=5
  vad : Inport  Port=6
  vaq : Inport  Port=7
  iad : Inport  Port=8
  iaq : Inport  Port=9
  Gain : Gain  Gain=2./Cf_pu
  PI Vc2 : Subsystem
  Product{1..2,5..6} (4 alike) : Product
  Sum : Sum  Inputs=|+-
  Sum1 : Sum  Inputs=|++
  Sum2 : Sum  Inputs=+-|
  Sum4 : Sum  Inputs=|++
  Vc : Integrator  InitialCondition=op_DFIG.Vc_control_Vc
  iad_ref : Outport  VectorParamsAs1DForOutWhenUnconnected=off
  wires:
  Sum1/1 -> Sum2/2
  Product1/1 -> Sum1/1
  Product2/1 -> Sum1/2
  vad/1 -> Product1/1
  vaq/1 -> Product2/1
  iaq/1 -> Product2/2
  iad/1 -> Product1/2
  Sum4/1 -> Sum2/1
  ird/1 -> Product5/2
  irq/1 -> Product6/2
  vrq/1 -> Product6/1
  vrd/1 -> Product5/1
  Product6/1 -> Sum4/2
  Product5/1 -> Sum4/1
  Sum/1 -> PI Vc2/1(in)
  PI Vc2/1(out) -> iad_ref/1
  Sum2/1 -> Gain/1
  Vc/1 -> Sum/2
  Gain/1 -> Vc/1
  Vc_2_ref/1 -> Sum/1

== system lib_AC_DFIG/DFIG/connect ==
  id : Inport
  iq : Inport  Port=2
  connect : Inport  Port=3
  Switch : Switch  Criteria=u2 > Threshold  ZeroCross=off  SaturateOnIntegerOverflow=off  InputSameDT=off
  Switch1 : Switch  Criteria=u2 > Threshold  ZeroCross=off  SaturateOnIntegerOverflow=off  InputSameDT=off
  Zero1 : Constant  Value=0  VectorParams1D=off  OutDataTypeStr=Inherit: Inherit via back propagation
  Zero2 : Constant  Value=0  VectorParams1D=off  OutDataTypeStr=Inherit: Inherit via back propagation
  id_real : Outport
  iq_real : Outport  Port=2
  connected : Outport  Port=3  OutDataTypeStr=boolean
  wires:
  Switch/1 -> id_real/1
  Zero1/1 -> Switch/3
  id/1 -> Switch/1
  connect/1 -> connected/1, Switch1/2, Switch/2
  Switch1/1 -> iq_real/1
  iq/1 -> Switch1/1
  Zero2/1 -> Switch1/3

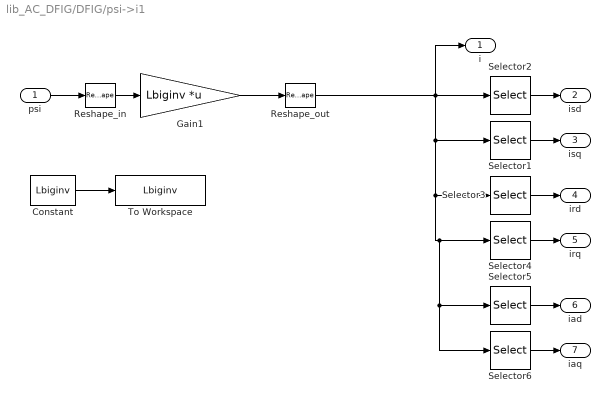
== system lib_AC_DFIG/DFIG/psi->i1 ==
  psi : Inport
  Constant : Constant  Value=Lbiginv
  Gain1 : Gain  Gain=Lbiginv  Multiplication=Matrix(K*u)
  Reshape_in : Reshape  OutputDimensionality=Column vector (2-D)  OutputDimensions=-1
  Reshape_out : Reshape  OutputDimensionality=Customize  OutputDimensions=[6*length(block_buses), 1]
  Selector1 : Selector  NumberOfDimensions=2  InputPortWidth=9  IndexOptions=Index vector (dialog),Select all  Indices=2,1  OutputSizes=1,1
  Selector2 : Selector  NumberOfDimensions=2  InputPortWidth=9  IndexOptions=Index vector (dialog),Select all  Indices=1,1  OutputSizes=1,1
  Selector3 : Selector  NumberOfDimensions=2  InputPortWidth=9  IndexOptions=Index vector (dialog),Select all  Indices=3,1  OutputSizes=1,1
  Selector4 : Selector  NumberOfDimensions=2  InputPortWidth=9  IndexOptions=Index vector (dialog),Select all  Indices=4,1  OutputSizes=1,1
  Selector5 : Selector  NumberOfDimensions=2  InputPortWidth=9  IndexOptions=Index vector (dialog),Select all  Indices=5,1  OutputSizes=1,1
  Selector6 : Selector  NumberOfDimensions=2  InputPortWidth=9  IndexOptions=Index vector (dialog),Select all  Indices=6,1  OutputSizes=1,1
  To Workspace : ToWorkspace  VariableName=Lbiginv  SaveFormat=Timeseries  SampleTime=-1
      settings: MaxDataPoints=1
  i : Outport  VectorParamsAs1DForOutWhenUnconnected=off
  isd : Outport  Port=2  VectorParamsAs1DForOutWhenUnconnected=off
  isq : Outport  Port=3  VectorParamsAs1DForOutWhenUnconnected=off
  ird : Outport  Port=4  VectorParamsAs1DForOutWhenUnconnected=off
  irq : Outport  Port=5  VectorParamsAs1DForOutWhenUnconnected=off
  iad : Outport  Port=6  VectorParamsAs1DForOutWhenUnconnected=off
  iaq : Outport  Port=7  VectorParamsAs1DForOutWhenUnconnected=off
  wires:
  Reshape_in/1 -> Gain1/1
  Gain1/1 -> Reshape_out/1
  psi/1 -> Reshape_in/1
  Constant/1 -> To Workspace/1
  Selector2/1 -> isd/1
  Selector1/1 -> isq/1
  Selector3/1 -> ird/1
  Selector4/1 -> irq/1
  Selector5/1 -> iad/1
  Selector6/1 -> iaq/1
  Reshape_out/1 -> Selector6/1, Selector5/1, Selector4/1, Selector3/1, Selector1/1, i/1, Selector2/1

== system lib_AC_DFIG/DFIG/trim_output ==
  id : Inport
  iq : Inport  Port=2
  vd : Inport  Port=3
  vq : Inport  Port=4
  Out1 : Outport
  Out2 : Outport  Port=2
  Out3 : Outport  Port=3
  Out4 : Outport  Port=4
  wires:
  id/1 -> Out1/1
  vq/1 -> Out4/1
  vd/1 -> Out3/1
  iq/1 -> Out2/1

== system lib_AC_DFIG/DFIG/w_ref_TF ==
  in : Inport
  Gain : Gain  Gain=1./T_s
  Sum4 : Sum  Inputs=|+-
  x_a : Integrator  InitialCondition=op_DFIG.w_ref_TF_x_a
  out : Outport
  wires:
  Gain/1 -> x_a/1
  Sum4/1 -> Gain/1
  x_a/1 -> out/1, Sum4/2
  in/1 -> Sum4/1

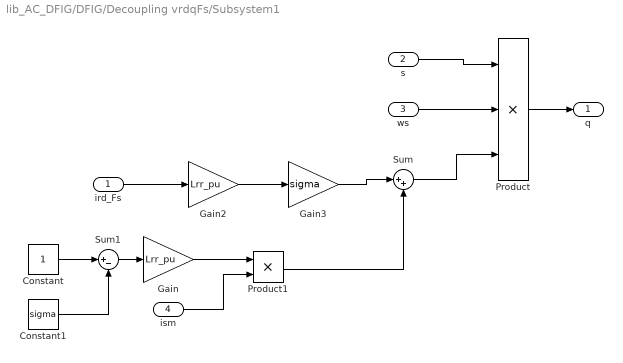
== system lib_AC_DFIG/DFIG/Decoupling vrdqFs/Subsystem1 ==
  ird_Fs : Inport
  s : Inport  Port=2
  ws : Inport  Port=3
  ism : Inport  Port=4
  Constant : Constant
  Constant1 : Constant  Value=sigma
  Gain : Gain  Gain=Lrr_pu
  Gain2 : Gain  Gain=Lrr_pu
  Gain3 : Gain  Gain=sigma
  Product : Product  Inputs=3
  Product1 : Product
  Sum : Sum  Inputs=|++
  Sum1 : Sum  Inputs=|+-
  q : Outport
  wires:
  Product/1 -> q/1
  ird_Fs/1 -> Gain2/1
  ws/1 -> Product/2
  Product1/1 -> Sum/2
  s/1 -> Product/1
  Gain/1 -> Product1/1
  Gain2/1 -> Gain3/1
  Gain3/1 -> Sum/1
  Constant/1 -> Sum1/1
  Constant1/1 -> Sum1/2
  Sum1/1 -> Gain/1
  ism/1 -> Product1/2
  Sum/1 -> Product/3

== system lib_AC_DFIG/DFIG/Decoupling vrdqFs/Subsystem2 ==
  irq_Fs : Inport
  s : Inport  Port=2
  ws : Inport  Port=3
  Constant : Constant  Value=sigma
  Display : Display
  Gain : Gain  Gain=Lrr_pu
  Gain1 : Gain  Gain=sigma
  Product : Product
  Product1 : Product
  d : Outport
  wires:
  Gain/1 -> Gain1/1
  Product/1 -> Gain/1
  s/1 -> Product/1
  Gain1/1 -> Product1/2
  ws/1 -> Product/2
  irq_Fs/1 -> Product1/1
  Product1/1 -> d/1
  Constant/1 -> Display/1

== system lib_AC_DFIG/DFIG/GSC Control/PI Estator Current d ==
  in : Inport
  Gain : Gain  Gain=Kp_ia
  Gain1 : Gain  Gain=Ki_ia
  Sum : Sum  Inputs=++|
  xa2 : Integrator  InitialCondition=op_DFIG.GSC_Control_PI_Estator_Current_d_xa2
  out : Outport  VectorParamsAs1DForOutWhenUnconnected=off
  wires:
  xa2/1 -> Sum/2
  Gain/1 -> Sum/1
  in/1 -> Gain1/1, Gain/1
  Sum/1 -> out/1
  Gain1/1 -> xa2/1

== system lib_AC_DFIG/DFIG/GSC Control/PI Estator Current q ==
  in : Inport
  Gain : Gain  Gain=Kp_ia
  Gain1 : Gain  Gain=Ki_ia
  Sum : Sum  Inputs=++|
  xa1 : Integrator  InitialCondition=op_DFIG.GSC_Control_PI_Estator_Current_q_xa1
  out : Outport  VectorParamsAs1DForOutWhenUnconnected=off
  wires:
  Gain1/1 -> xa1/1
  Sum/1 -> out/1
  in/1 -> Gain/1, Gain1/1
  Gain/1 -> Sum/1
  xa1/1 -> Sum/2

== system lib_AC_DFIG/DFIG/GSC Control/Subsystem1 ==
  ws : Inport
  vaq' : Inport  Port=2
  vsq : Inport  Port=3
  iad : Inport  Port=4
  Gain1 : Gain  Gain=La_pu
  Product1 : Product
  Sum4 : Sum  Inputs=-|+|-  InputSameDT=on  SaturateOnIntegerOverflow=on  OutDataTypeStr=Inherit: Same as first input
  vadq : Outport
  wires:
  iad/1 -> Product1/2
  Gain1/1 -> Product1/1
  vaq'/1 -> Sum4/1
  Sum4/1 -> vadq/1  "vadq"
  Product1/1 -> Sum4/3
  ws/1 -> Gain1/1
  vsq/1 -> Sum4/2

== system lib_AC_DFIG/DFIG/GSC Control/Subsystem3 ==
  vad' : Inport
  vd : Inport  Port=2
  iaq : Inport  Port=3
  ws : Inport  Port=4
  Gain1 : Gain  Gain=La_pu
  Product1 : Product
  Sum4 : Sum  Inputs=-|+|+  InputSameDT=on  SaturateOnIntegerOverflow=on  OutDataTypeStr=Inherit: Same as first input
  vad : Outport
  wires:
  iaq/1 -> Product1/2
  ws/1 -> Gain1/1
  Product1/1 -> Sum4/3
  Sum4/1 -> vad/1  "vadq"
  vd/1 -> Sum4/2
  vad'/1 -> Sum4/1
  Gain1/1 -> Product1/1

== system lib_AC_DFIG/DFIG/RSC Control/PI Rotor Current d ==
  in : Inport
  Gain : Gain  Gain=Kp_ir
  Gain1 : Gain  Gain=Ki_ir
  Sum : Sum  Inputs=++|
  xr1 : Integrator  InitialCondition=op_DFIG.RSC_Control_PI_Rotor_Current_d_xr1
  out : Outport  VectorParamsAs1DForOutWhenUnconnected=off
  wires:
  Gain1/1 -> xr1/1
  Sum/1 -> out/1
  in/1 -> Gain/1, Gain1/1
  Gain/1 -> Sum/1
  xr1/1 -> Sum/2

== system lib_AC_DFIG/DFIG/RSC Control/PI Rotor Current q ==
  in : Inport
  Gain : Gain  Gain=Kp_ir
  Gain1 : Gain  Gain=Ki_ir
  Sum : Sum  Inputs=++|
  xr2 : Integrator  InitialCondition=op_DFIG.RSC_Control_PI_Rotor_Current_q_xr2
  out : Outport  VectorParamsAs1DForOutWhenUnconnected=off
  wires:
  xr2/1 -> Sum/2
  Gain/1 -> Sum/1
  in/1 -> Gain1/1, Gain/1
  Sum/1 -> out/1
  Gain1/1 -> xr2/1

== system lib_AC_DFIG/DFIG/Slip/PI Slip ==
  in : Inport
  Gain : Gain  Gain=Kp_s
  Gain1 : Gain  Gain=Ki_s
  Sum : Sum  Inputs=++|
  xr3 : Integrator  InitialCondition=op_DFIG.Slip_PI_Slip_xr3  UpperSaturationLimit=1.01  LowerSaturationLimit=0.99
  out : Outport  VectorParamsAs1DForOutWhenUnconnected=off
  wires:
  xr3/1 -> Sum/2
  Gain/1 -> Sum/1
  in/1 -> Gain1/1, Gain/1
  Sum/1 -> out/1
  Gain1/1 -> xr3/1

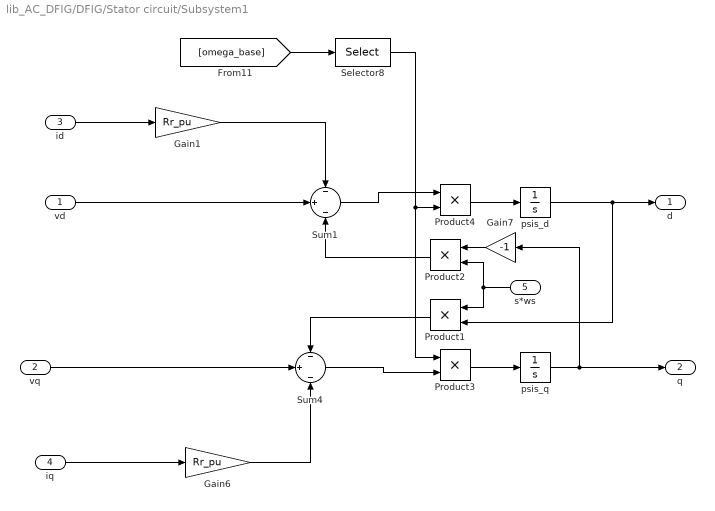
== system lib_AC_DFIG/DFIG/Stator circuit/Subsystem1 ==
  vd : Inport
  vq : Inport  Port=2
  id : Inport  Port=3
  iq : Inport  Port=4
  s*ws : Inport  Port=5
  Gain1 : Gain  Gain=Rr_pu
  Gain6 : Gain  Gain=Rr_pu
  Gain7 : Gain  Gain=-1
  Product{1..4} (4 alike) : Product
  Selector8 : Selector  InputPortWidth=length(fref.ref_units)  IndexOptions=Index vector (dialog)  Indices=block_fref  OutputSizes=1
  Sum1 : Sum  Inputs=-|+|-  InputSameDT=on  SaturateOnIntegerOverflow=on  OutDataTypeStr=Inherit: Same as first input
  Sum4 : Sum  Inputs=-|+|-  InputSameDT=on  SaturateOnIntegerOverflow=on  OutDataTypeStr=Inherit: Same as first input
  psis_d : Integrator  InitialCondition=op_DFIG.Stator_circuit_Subsystem1_psis_d
  psis_q : Integrator  InitialCondition=op_DFIG.Stator_circuit_Subsystem1_psis_q
  d : Outport
  q : Outport  Port=2
  wires:
  Product1/1 -> Sum4/1
  s*ws/1 -> Product1/1, Product2/2
  Gain6/1 -> Sum4/3
  Product3/1 -> psis_q/1
  Sum1/1 -> Product4/1
  psis_d/1 -> Product1/2, d/1
  Sum4/1 -> Product3/2
  Product4/1 -> psis_d/1
  Gain1/1 -> Sum1/1
  Gain7/1 -> Product2/1
  id/1 -> Gain1/1
  Product2/1 -> Sum1/3
  psis_q/1 -> q/1, Gain7/1
  iq/1 -> Gain6/1
  vd/1 -> Sum1/2
  vq/1 -> Sum4/2
  Selector8/1 -> Product3/1, Product4/2
  [omega_base] -> Selector8/1

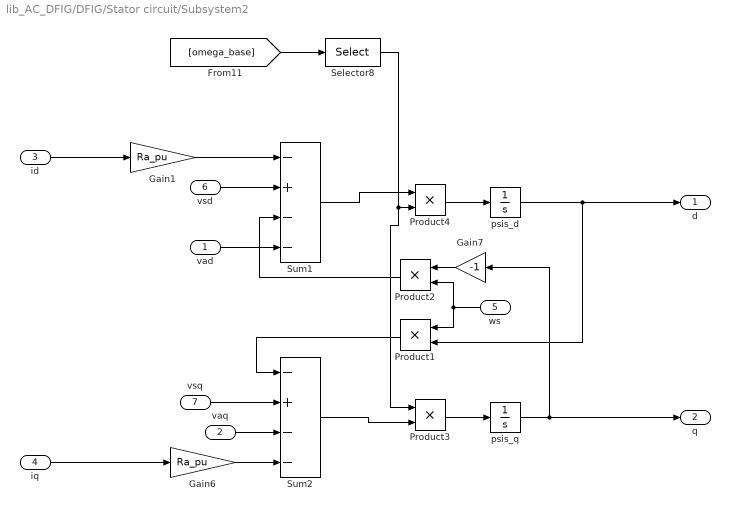
== system lib_AC_DFIG/DFIG/Stator circuit/Subsystem2 ==
  vad : Inport
  vaq : Inport  Port=2
  id : Inport  Port=3
  iq : Inport  Port=4
  ws : Inport  Port=5
  vsd : Inport  Port=6
  vsq : Inport  Port=7
  Gain1 : Gain  Gain=Ra_pu
  Gain6 : Gain  Gain=Ra_pu
  Gain7 : Gain  Gain=-1
  Product{1..4} (4 alike) : Product
  Selector8 : Selector  InputPortWidth=length(fref.ref_units)  IndexOptions=Index vector (dialog)  Indices=block_fref  OutputSizes=1
  Sum1 : Sum  Inputs=-|+|-|-  InputSameDT=on  SaturateOnIntegerOverflow=on  OutDataTypeStr=Inherit: Same as first input
  Sum2 : Sum  Inputs=-|+|-|-  InputSameDT=on  SaturateOnIntegerOverflow=on  OutDataTypeStr=Inherit: Same as first input
  psis_d : Integrator  InitialCondition=op_DFIG.Stator_circuit_Subsystem2_psis_d
  psis_q : Integrator  InitialCondition=op_DFIG.Stator_circuit_Subsystem2_psis_q
  d : Outport
  q : Outport  Port=2
  wires:
  iq/1 -> Gain6/1
  psis_q/1 -> Gain7/1, q/1
  Product2/1 -> Sum1/3
  id/1 -> Gain1/1
  Gain7/1 -> Product2/1
  Gain1/1 -> Sum1/1
  Product4/1 -> psis_d/1
  Sum2/1 -> Product3/2
  psis_d/1 -> Product1/2, d/1
  Sum1/1 -> Product4/1
  Product3/1 -> psis_q/1
  ws/1 -> Product2/2, Product1/1
  vsd/1 -> Sum1/2
  vad/1 -> Sum1/4
  Gain6/1 -> Sum2/4
  vsq/1 -> Sum2/2
  Product1/1 -> Sum2/1
  vaq/1 -> Sum2/3
  Selector8/1 -> Product3/1, Product4/2
  [omega_base] -> Selector8/1

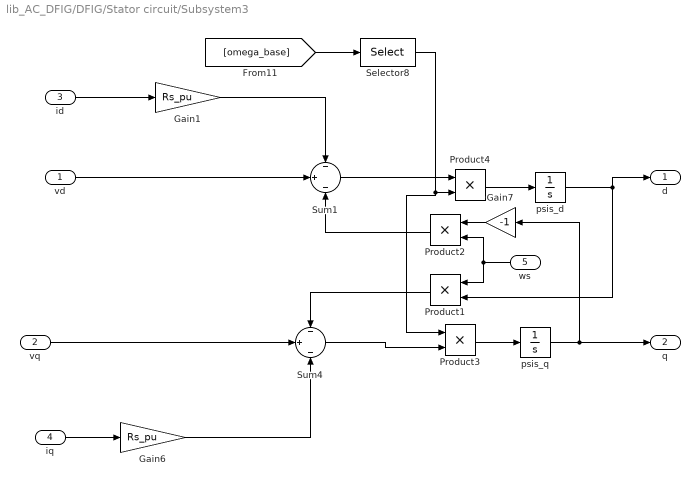
== system lib_AC_DFIG/DFIG/Stator circuit/Subsystem3 ==
  vd : Inport
  vq : Inport  Port=2
  id : Inport  Port=3
  iq : Inport  Port=4
  ws : Inport  Port=5
  Gain1 : Gain  Gain=Rs_pu
  Gain6 : Gain  Gain=Rs_pu
  Gain7 : Gain  Gain=-1
  Product{1..4} (4 alike) : Product
  Selector8 : Selector  InputPortWidth=length(fref.ref_units)  IndexOptions=Index vector (dialog)  Indices=block_fref  OutputSizes=1
  Sum1 : Sum  Inputs=-|+|-  InputSameDT=on  SaturateOnIntegerOverflow=on  OutDataTypeStr=Inherit: Same as first input
  Sum4 : Sum  Inputs=-|+|-  InputSameDT=on  SaturateOnIntegerOverflow=on  OutDataTypeStr=Inherit: Same as first input
  psis_d : Integrator  InitialCondition=op_DFIG.Stator_circuit_Subsystem3_psis_d
  psis_q : Integrator  InitialCondition=op_DFIG.Stator_circuit_Subsystem3_psis_q
  d : Outport
  q : Outport  Port=2
  wires:
  vq/1 -> Sum4/2
  vd/1 -> Sum1/2
  iq/1 -> Gain6/1
  psis_q/1 -> q/1, Gain7/1
  Product2/1 -> Sum1/3
  id/1 -> Gain1/1
  Gain7/1 -> Product2/1
  Product4/1 -> psis_d/1
  Sum4/1 -> Product3/2
  psis_d/1 -> d/1, Product1/2
  Sum1/1 -> Product4/1
  Product3/1 -> psis_q/1
  ws/1 -> Product2/2, Product1/1
  Product1/1 -> Sum4/1
  Gain1/1 -> Sum1/1
  Gain6/1 -> Sum4/3
  Selector8/1 -> Product3/1, Product4/2
  [omega_base] -> Selector8/1

== system lib_AC_DFIG/DFIG/Vc control/PI Vc2 ==
  in : Inport
  Gain : Gain  Gain=Kp_vc2
  Gain1 : Gain  Gain=Ki_vc2
  Sum : Sum  Inputs=++|
  xa3 : Integrator  InitialCondition=op_DFIG.Vc_control_PI_Vc2_xa3
  out : Outport  VectorParamsAs1DForOutWhenUnconnected=off
  wires:
  Gain1/1 -> xa3/1
  Sum/1 -> out/1
  in/1 -> Gain/1, Gain1/1
  Gain/1 -> Sum/1
  xa3/1 -> Sum/2
